simulink model "scheme_L2"  (R2026b)
settings: Solver=ode45  StopTime=10
settings Model: Creator=User  LastModifiedBy=User
settings DebuggingCC: AlgebraicLoopMsg=none

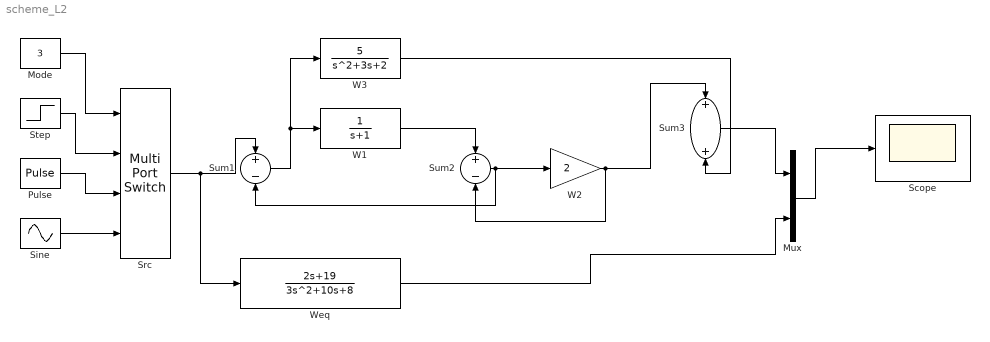
== system scheme_L2 ==
  Mode : Constant  Value=3
  Mux : Mux  Inputs=2
  Pulse : DiscretePulseGenerator  PulseType=Time based  Period=10
  Scope : Scope
      settings: ActiveDisplayYMinimum=-0.017765690209550961  ActiveDisplayYMaximum=0.15989121188595867
  Sine : Sin  SampleTime=0
  Src : MultiPortSwitch  SaturateOnIntegerOverflow=off  InputSameDT=off
  Step : Step  Time=0  SampleTime=0
  Sum1 : Sum  Inputs=+-
  Sum2 : Sum  Inputs=+-
  Sum3 : Sum  Inputs=+|+
  W1 : TransferFcn  Denominator=[1 1]
  W2 : Gain  Gain=2
  W3 : TransferFcn  Numerator=[5]  Denominator=[1 3 2]
  Weq : TransferFcn  Numerator=[2 19]  Denominator=[3 10 8]
  wires:
  Mode/1 -> Src/1
  Step/1 -> Src/2
  Pulse/1 -> Src/3
  Sine/1 -> Src/4
  Src/1 -> Sum1/1, Weq/1
  Sum1/1 -> W1/1, W3/1
  W1/1 -> Sum2/1
  Sum2/1 -> W2/1, Sum1/2
  W2/1 -> Sum2/2, Sum3/1
  W3/1 -> Sum3/2
  Sum3/1 -> Mux/1
  Weq/1 -> Mux/2
  Mux/1 -> Scope/1
